simulink model "DDMR_Simscape_PID_Motor"  (R2024b)
settings: Solver=ode23t  StartTime=0.0  StopTime=3  FixedStep=0.005  RelTol=1e-3
values from neighbouring files (symbols this model uses):
  L = 0.2    [LQR.m]    (also in Track.m; Track2.m)
  L_f = 0.2    [LQR.m]    (also in Track.m; Track2.m)
  line_width = 0.03    [LQR.m]    (also in Track.m; Track2.m)
  N = size(pts, 1)    [Track2.m]
  R = 0.05    [LQR.m]    (also in Track.m; Track2.m)
  track_pts = [2*cos(linspace(0, 2*pi, 1000)'), 2*sin(linspace(0, 2*pi, 1000)').*cos(linspace(0, 2*pi, 1000)')]    [LQR.m]    (also in Track.m; Track2.m = [track_pts; segments{i}])
  W_spread = 0.15    [LQR.m]    (also in Track.m; Track2.m)
undefined symbols (not defined in the file or in its folder): X, Y, Z
libraries: sm_lib x22, fl_lib x8, nesl_utility x8, slpidlib x4, ee_lib x2
(part 2 of 2)

== matlab function DDMR_Simscape_PID_Motor/Inverse_Kinematiks 1 ==
  data: v input; omega_L output; omega input; R input; L input; omega_R output
function [omega_L, omega_R] = inverse_kinematics(v, omega, R, L)
    % Calculate linear velocity of each wheel (m/s)
    v_L = v - (omega * L / 2);
    v_R = v + (omega * L / 2);

    % Convert linear velocity to angular velocity (rad/s)
    omega_L = v_L / R;
    omega_R = v_R / R;
end

== matlab function DDMR_Simscape_PID_Motor/MATLAB Function1 ==
  settings: updateMethod=DISCRETE
  data: sensor_readings input; error output
function error = calculate_error(sensor_readings)
    % Assign weights to the 6 sensors: far left is positive error, far right is negative
    weights = [5, 3, 1, -1, -3, -5]; 
    
    persistent prev_error;
    if isempty(prev_error)
        prev_error = 0;
    end
    
    if sum(sensor_readings) == 0
        % Track lost: rely on memory to keep steering back toward the line
        error = prev_error; 
    else
        % Track found: calculate new error and update memory
        error = sum(sensor_readings .* weights);
        prev_error = error; 
    end
end
